simulink model "Pay_load"  (R2025a)
settings: Solver=ode4  StartTime=0.0  StopTime=1  FixedStep=0.001  RelTol=1e-3
values from neighbouring files (symbols this model uses):
  angle1_init = [0;0;0.3]    [param.m]
  angle2_init = [0;0;0.3]    [param.m]
  angle3_init = [0;0;0.3]    [param.m]
  angle4_init = [0;0;0.3]    [param.m]
  joint_matrix = [r1; r2; r3; r4]    [param.m]
  m1 = 1    [param.m]
  m2 = 1    [param.m]
  m3 = 1    [param.m]
  m4 = 1    [param.m]
  mL = 2    [param.m]
  P = block.DialogPrm(1).Data    [Load_dynamic.m]    (also in param.m = struct())
  p1_init = pL_init + RL_init*r1 - l1*e1    [param.m]
  p2_init = pL_init + RL_init*r2 - l2*e2    [param.m]
  p3_init = pL_init + RL_init*r3 - l3*e3    [param.m]
  p4_init = pL_init + RL_init*r4 - l4*e4    [param.m]
  r1 = [ 0.25; -0.20; -0.45]    [param.m]
  r2 = [-0.50; -0.40; -0.15]    [param.m]
  r3 = [-0.50;  0.40;  0.15]    [param.m]
  r4 = [ 0.50;  0.40;  0.00]    [param.m]
  xL_init = [pL_init; vL_init; angle_L_init; omega_L_init]    [param.m]
(part 2 of 3)

== matlab function Pay_load/PayLoad Controller/Subsystem/Adaptive Law (eq. 31) ==
  data: z4L input; delta_2L_dot output; delta_2L input
function delta_2L_dot = fcn(z4L, delta_2L)

    n_delta2L = 0.25; sigma_delta2L = 0.1; epsilon_L = 0.1;

    delta_2L_dot = n_delta2L*norm(z4L)^2/sqrt(norm(z4L)^2 + epsilon_L^2) - sigma_delta2L*delta_2L;

end

== matlab function Pay_load/PayLoad Controller/MATLAB Function3 ==
  data: angle_dL input; R_dL output
function R_dL = fcn(angle_dL)

    phi_dL = angle_dL(1); theta_dL = angle_dL(2); psi_dL = angle_dL(3);

    R_dL = [cos(theta_dL)*cos(psi_dL), sin(phi_dL)*sin(theta_dL)*cos(psi_dL) - cos(phi_dL)*sin(psi_dL), cos(phi_dL)*sin(theta_dL)*cos(psi_dL) + sin(phi_dL)*sin(psi_dL);
            cos(theta_dL)*sin(psi_dL), sin(phi_dL)*sin(theta_dL)*sin(psi_dL) + cos(phi_dL)*cos(psi_dL), cos(phi_dL)*sin(theta_dL)*sin(psi_dL) - sin(phi_dL)*cos(psi_dL);
            -sin(theta_dL)           , sin(phi_dL)*cos(theta_dL)                                      , cos(phi_dL)*cos(theta_dL)];

    
end

== matlab function Pay_load/PayLoad Controller/Equation (35) ==
  data: u input; cable_tension output; joint_matrix parameter
function cable_tension = fcn(u, joint_matrix)

    r1 = joint_matrix(1:3, 1);
    r2 = joint_matrix(4:6, 1);
    r3 = joint_matrix(7:9, 1);
    r4 = joint_matrix(10:12, 1);


    S = @(r) [0, -r(3), r(2);
              r(3), 0, -r(1);
              -r(2), r(1), 0];

    P = [eye(3), eye(3), eye(3), eye(3);
         S(r1) , S(r2) , S(r3) , S(r4)];

    P_inv = P' / (P * P');

    cable_tension = P_inv * u;

end

== matlab function Pay_load/PayLoad Controller/Equation (77) ==
  data: angle_L_dot input; Psi_L input; Psi_L_dot input; alpha_angle_L_dot input; alpha_angle_L input; sq_L output
function sq_L = fcn(angle_L_dot, Psi_L, Psi_L_dot, alpha_angle_L_dot, alpha_angle_L)

    S = @(r) [0, -r(3), r(2);
              r(3), 0, -r(1);
              -r(2), r(1), 0];
    
    sq_L = norm(Psi_L)*(norm(Psi_L*alpha_angle_L_dot + Psi_L_dot*alpha_angle_L) + norm(S(Psi_L*angle_L_dot))*norm(Psi_L*alpha_angle_L));

end

== matlab function Pay_load/UAV1 Controller/Subsystem1/Position Controller/Equation (8) ==
  data: ei input; dei output
function dei = fcn(ei)

    dei = norm(ei);

end

== matlab function Pay_load/Subsystem/UAV1/MATLAB Function ==
  data: a_free input; p_ddot output; fCableWorld input; m parameter
function p_ddot = UAV_Acceleration(a_free, fCableWorld, m)
%#codegen
% fCableWorld: luc day THUC tac dung len UAV, he the gioi.

assert(m > 0);

p_ddot = a_free + fCableWorld/m;
end

== matlab function Pay_load/UAV1 Controller/Subsystem1/Position Controller/Equation (15) ==
  data: dei input; eta_e1 output; t input; d_eta_d_dei output
function [eta_e1, d_eta_d_dei]= fcn(dei, t)
    
    eta_e1 = 0;

    Omega_dHi = (7.8 - 0.2)*exp(-0.4*t) + 0.2;

    eta_e1 = (Omega_dHi*dei)/(Omega_dHi - dei);

    d_eta_d_dei = Omega_dHi^2/(Omega_dHi - dei)^2;

end

== matlab function Pay_load/UAV1 Controller/Subsystem1/Position Controller/MATLAB Function ==
  data: dij input; t input; d_eij output; vij input; eta_eij output; d_eta_d_deij output
function [d_eij, eta_eij, d_eta_d_deij]   = fcn(dij, t, vij)

    d_eij = zeros(3,1);
    eta_eij = zeros(3,1);
    d_eta_d_deij = zeros(3,1);

    d12 = dij(1); d13 = dij(2); d14 = dij(3);
    v12 = vij(1); v13 = vij(2); v14 = vij(3);


    Omega_Hij = (2 - 0.1)*exp(-0.1*t) + 0.1;
    Omega_Wij = (1.8 - 0.1)*exp(-0.15*t) + 0.1;

    A = @(d_eij) (Omega_Hij*Omega_Wij*(Omega_Hij*Omega_Wij + d_eij^2))/((Omega_Hij - d_eij)^2*(Omega_Wij + d_eij)^2);

    d_e12 = d12 - v12; d_e13 = d13 - v13; d_e14 = d14 - v14;

    eta_e12 = (Omega_Hij*Omega_Wij*d_e12)/((Omega_Hij - d_e12) * (Omega_Wij + d_e12));
    eta_e13 = (Omega_Hij*Omega_Wij*d_e13)/((Omega_Hij - d_e13) * (Omega_Wij + d_e13));
    eta_e14 = (Omega_Hij*Omega_Wij*d_e14)/((Omega_Hij - d_e14) * (Omega_Wij + d_e14));

    d_eij = [d_e12; d_e13; d_e14];
    eta_eij = [eta_e12; eta_e13; eta_e14];

    d_eta_d_de12 = A(d_e12); d_eta_d_de13 = A(d_e13); d_eta_d_de14 = A(d_e14);

    d_eta_d_deij = [d_eta_d_de12; d_eta_d_de13; d_eta_d_de14];
    
end

== matlab function Pay_load/UAV1 Controller/Subsystem1/Position Controller/Equation (10) ==
  data: e12 input; dij output; e13 input; e14 input
function dij = fcn(e12, e13, e14)

    dij = zeros(3,1);

    d12 = norm(e12);
    d13 = norm(e13);
    d14 = norm(e14);


    dij = [d12; d13; d14];
end

== matlab function Pay_load/UAV1 Controller/Subsystem1/Position Controller/Equation (9) ==
  data: e_d12 input; vij output; e_d13 input; e_d14 input
function vij = fcn(e_d12, e_d13, e_d14)

    vij = zeros(3,1);

    v12 = norm(e_d12);
    v13 = norm(e_d13);
    v14 = norm(e_d14);

    vij = [v12; v13; v14];

end

== matlab function Pay_load/Subsystem/UAV1/MATLAB Function2 ==
  data: angle input; angle_dot output; omega input
function angle_dot = fcn(angle, omega)

    angle_dot = zeros(3,1);

    phi = angle(1); theta = angle(2);

    Gamma = [1, sin(phi)*tan(theta), cos(phi)*tan(theta);
            0, cos(phi), -sin(phi);
            0, sin(phi)/cos(theta), cos(phi)/cos(theta)];

    angle_dot = Gamma * omega;

end

== matlab function Pay_load/Subsystem1/UAV2/MATLAB Function2 ==
  data: angle input; angle_dot output; omega input
function angle_dot = fcn(angle, omega)

    angle_dot = zeros(3,1);

    phi = angle(1); theta = angle(2);

    Gamma = [1, sin(phi)*tan(theta), cos(phi)*tan(theta);
            0, cos(phi), -sin(phi);
            0, sin(phi)/cos(theta), cos(phi)/cos(theta)];

    angle_dot = Gamma * omega;

end

== matlab function Pay_load/Subsystem2/UAV3/MATLAB Function2 ==
  data: angle input; angle_dot output; omega input
function angle_dot = fcn(angle, omega)

    angle_dot = zeros(3,1);

    phi = angle(1); theta = angle(2);

    Gamma = [1, sin(phi)*tan(theta), cos(phi)*tan(theta);
            0, cos(phi), -sin(phi);
            0, sin(phi)/cos(theta), cos(phi)/cos(theta)];

    angle_dot = Gamma * omega;

end

== matlab function Pay_load/Subsystem3/UAV4/MATLAB Function2 ==
  data: angle input; angle_dot output; omega input
function angle_dot = fcn(angle, omega)

    angle_dot = zeros(3,1);

    phi = angle(1); theta = angle(2);

    Gamma = [1, sin(phi)*tan(theta), cos(phi)*tan(theta);
            0, cos(phi), -sin(phi);
            0, sin(phi)/cos(theta), cos(phi)/cos(theta)];

    angle_dot = Gamma * omega;

end

== matlab function Pay_load/UAV1 Controller/Subsystem1/Position Controller/MATLAB Function1 ==
  data: dei input; eta_ei input; d_eta_d_dei input; ei input; eij input; d_ij input; Ei output; eta_eij input; d_eta_d_eij input
function Ei = fcn(dei, eta_ei, d_eta_d_dei, ei, eij, d_ij, eta_eij, d_eta_d_eij)

    Ei = zeros(3,1);

    A = d_eta_d_dei * sqrt(d_eta_d_dei) * ei;
    
    B = zeros(3,1);
    for i = 1:3
        B = B + 2*eta_eij(i)*d_eta_d_eij(i)*eij(((i-1)*3+1):(i*3),1)/d_ij(i);
    end

    Ei = A + B;

end

== matlab function Pay_load/UAV1 Controller/Subsystem1/Position Controller/Equation (38) ==
  data: ei input; dei input; eta_ei input; d_eta_d_dei input; alpha_pi output; Ei input; eta_eij input; pd_dot input; t input; e_dij input; e_dij_dot input; vij input; d_eij input; d_eta_d_deij input
function alpha_pi = fcn(ei, dei, eta_ei, d_eta_d_dei, Ei, eta_eij, pd_dot, t, e_dij, e_dij_dot, vij, d_eij, d_eta_d_deij)

    alpha_pi = zeros(3,1);

    Kei = 3.15; Keij = 0.45;
    
    %% Eta_i
    Omega_dHi = (7.8 - 0.2)*exp(-0.4*t) + 0.2;
    Omega_dHi_dot = -0.4*7.6*exp(-0.4*t);
    d_eta_d_Omega_dHi = -dei^2/(Omega_dHi - dei)^2;

    h = Omega_dHi;
    hdot = Omega_dHi_dot;
    gap = h - dei;

    assert(gap > 1e-9, ...
        'Sai so vi tri da cham hoac vuot bien.');

    Gi = (h/gap)^3 * ei;

    eta_Eta_i = Gi.'*pd_dot ...
                + eta_ei*(dei^2/gap^2)*hdot;
    
    
    %% Eta_eij
    Omega_Hij = (2 - 0.1)*exp(-0.1*t) + 0.1;
    Omega_Wij = (1.8 - 0.1)*exp(-0.15*t) + 0.1;

    Omega_Hij_dot = -0.1*1.9*exp(-0.1*t);
    Omega_Wij_dot = -0.15*1.7*exp(-0.15*t);

    C_Hij = @(d_eij) -Omega_Wij*d_eij^2/((Omega_Hij - d_eij)^2 * (Omega_Wij + d_eij));
    D_Wij = @(d_eij) Omega_Hij*d_eij^2/((Omega_Hij - d_eij)*(Omega_Wij + d_eij)^2);

    d_eta_d_Omega_Hij = [C_Hij(d_eij(1)); C_Hij(d_eij(2)); C_Hij(d_eij(3))];
    d_eta_d_Omega_Wij = [D_Wij(d_eij(1)); D_Wij(d_eij(2)); D_Wij(d_eij(3))];


    e_d12 = e_dij(1:3,1); e_d13 = e_dij(4:6,1); e_d14 = e_dij(7:9,1);
    e_d12_dot = e_dij_dot(1:3,1); e_d13_dot = e_dij_dot(4:6,1); e_d14_dot = e_dij_dot(7:9,1);
    
    Eta_e12 = d_eta_d_deij(1)/vij(1)*(e_d12(1)*e_d12_dot(1) + e_d12(2)*e_d12_dot(2) + e_d12(3)*e_d12_dot(3)) - (d_eta_d_Omega_Hij(1)*Omega_Hij_dot + d_eta_d_Omega_Wij(1)*Omega_Wij_dot);
    Eta_e13 = d_eta_d_deij(2)/vij(2)*(e_d13(1)*e_d13_dot(1) + e_d13(2)*e_d13_dot(2) + e_d13(3)*e_d13_dot(3)) - (d_eta_d_Omega_Hij(2)*Omega_Hij_dot + d_eta_d_Omega_Wij(2)*Omega_Wij_dot);
    Eta_e14 = d_eta_d_deij(3)/vij(3)*(e_d14(1)*e_d14_dot(1) + e_d14(2)*e_d14_dot(2) + e_d14(3)*e_d14_dot(3)) - (d_eta_d_Omega_Hij(3)*Omega_Hij_dot + d_eta_d_Omega_Wij(3)*Omega_Wij_dot);

    Eta_eij = [Eta_e12; Eta_e13; Eta_e14];

    B = 0;
    for i = 1:3
        B = B - Keij*eta_eij(i)^2 + eta_eij(i)*Eta_eij(i);
    end

    den = Ei.'*Ei;

    assert(den > 1e-12, ...
        'Phuong trinh 38 gan ky di: Ei gan bang 0.');

    alpha_pi = Ei/den * ...
            (-Kei*eta_ei^2 + eta_Eta_i + B);

end

== matlab function Pay_load/Subsystem1/UAV2/MATLAB Function ==
  data: a_free input; p_ddot output; fCableWorld input; m parameter
function p_ddot = UAV_Acceleration(a_free, fCableWorld, m)
%#codegen
% fCableWorld: luc day THUC tac dung len UAV, he the gioi.

assert(m > 0);

p_ddot = a_free + fCableWorld/m;
end

== matlab function Pay_load/UAV1 Controller/Subsystem1/Subsystem/MATLAB Function ==
  data: pi input; vi input; ui output; alpha_pi input; alpha_pi_dot input; Ei input; cable_tension input; delta_i input; rho_mi input; xL input; z2i output; ubar_i output; delta_i_dot output; rho_mi_dot output; m parameter; ri parameter
function [ui, z2i, ubar_i, delta_i_dot, rho_mi_dot] = ...
    Velocity_Control_41_44(pi, vi, alpha_pi, alpha_pi_dot, Ei, ...
                          cable_tension, delta_i, rho_mi, xL, m, ri)
    %#codegen
    % Vector inputs: 3x1
    % mi, delta_i, rho_mi: scalar
    
    K2i       = 3.15;
    epsilon_i = 0.1;
    
    n_delta     = 0.15;
    sigma_delta = 0.05;
    
    n_rho_m     = 0.1;
    sigma_rho_m = 0.01;
    
    assert(m > 0);
    
    ez = [0; 0; 1];
    
    z2i = vi - alpha_pi;
    z2_sq = z2i.' * z2i;
    
    %% Equation (42)
    pL = xL(1:3,1); phi_L = xL(7,1); theta_L = xL(8,1); psi_L = xL(9,1);

    RL = [cos(theta_L)*cos(psi_L), sin(phi_L)*sin(theta_L)*cos(psi_L) - cos(phi_L)*sin(psi_L), cos(phi_L)*sin(theta_L)*cos(psi_L) + sin(phi_L)*sin(psi_L);
          cos(theta_L)*sin(psi_L), sin(phi_L)*sin(theta_L)*sin(psi_L) + cos(phi_L)*cos(psi_L), cos(phi_L)*sin(theta_L)*sin(psi_L) - sin(phi_L)*cos(psi_L);
          -sin(theta_L), sin(phi_L)*cos(theta_L), cos(phi_L)*cos(theta_L)];

    qi = RL.'*(pL + RL*ri - pi)/norm(pL + RL*ri - pi);

    fCablePred_i = RL*qi*(cable_tension.'*qi);

    ubar_i = Ei - alpha_pi_dot ...
             + 9.81 * ez ...
             + K2i * z2i ...
             + delta_i * z2i / sqrt(z2_sq + epsilon_i^2) ...
             + fCablePred_i / m;
    
    %% Equation (41)
    ubar_sq = ubar_i.' * ubar_i;
    A = ubar_sq * rho_mi^2;
    
    ui = z2i * A / sqrt(z2_sq * A + epsilon_i^2);
    
    %% Equation (43)
    delta_i_dot = n_delta * z2_sq ...
                  / sqrt(z2_sq + epsilon_i^2) ...
                  - sigma_delta * delta_i;
    
    %% Equation (44)
    rho_mi_dot = n_rho_m * (z2i.' * ubar_i) ...
                - sigma_rho_m * rho_mi;

end

== matlab function Pay_load/UAV1 Controller/Subsystem1/Subsystem/MATLAB Function1 ==
  data: ui input; Fi output; psi_di input; angle_di_prev input; angle_di output; valid output
function [Fi, angle_di, valid] = ...
    Desired_Attitude_85_87(ui, psi_di, angle_di_prev)
%#codegen
% ui, angle_di_prev: 3x1
% psi_di, Fi: scalar
% valid: boolean

Fmin = 1e-8;

Fi = norm(ui);
angle_di = angle_di_prev;
valid = false;

% Khi ui gan 0, huong luc khong xac dinh.
% Giu goc dat truoc do, khong chia cho Fi.
if Fi <= Fmin
    return;
end

% Mien Euler bay thang dang su dung:
% |phi_di| < pi/2, |theta_di| < pi/2.
% assert(ui(3) > 0);

sphi = (ui(1)*sin(psi_di) ...
        - ui(2)*cos(psi_di)) / Fi;

% Chi chan sai so lam tron cua asin.
sphi = min(1.0, max(-1.0, sphi));

phi_di = asin(sphi);

theta_di = atan2( ...
    ui(1)*cos(psi_di) + ui(2)*sin(psi_di), ui(3));

angle_di = [phi_di; theta_di; psi_di];
valid = true;

end

== matlab function Pay_load/UAV1 Controller/Subsystem/MATLAB Function ==
  data: angle_i input; z3i output size=[3,1]; omega_i input; angle_di input; z4i output size=[3,1]; Gamma_i output size=[3,3]; alpha_angle_i output size=[3,1]; angle_i_dot output size=[3,1]; Psi_i output size=[3,3]; Psi_i_dot output size=[3,3]
function [z3i, z4i, Gamma_i, alpha_angle_i, angle_i_dot, Psi_i, Psi_i_dot] = ...
    Attitude_Error_56(angle_i, omega_i, angle_di)


    z3i = zeros(3,1);
    z4i = zeros(3,1);

    Gamma_i = zeros(3,3);

    alpha_angle_i = zeros(3,1);

    K3i = 0.75;
    nu_i = 0.5;
    
    phi   = angle_i(1);
    theta = angle_i(2);
    
    sp = sin(phi);
    cp = cos(phi);
    st = sin(theta);
    ct = cos(theta);
    
    assert(K3i > 0 && nu_i > 0);
    assert(abs(ct) > 1e-6);
    
    Gamma_i = [1, sp*st/ct, cp*st/ct;
               0, cp,       -sp;
               0, sp/ct,    cp/ct];
    
    Psi_i = [1, 0,   -st;
             0, cp,  sp*ct;
             0, -sp, cp*ct];
    
    angle_i_dot = Gamma_i * omega_i;
    
    z3i = angle_i - angle_di;
    
    k = K3i + 0.5*nu_i;
    alpha_angle_i = -k * z3i;
    
    z4i = angle_i_dot - alpha_angle_i;
    
    % Dao ham giai tich cua Psi_i
    phi_dot   = angle_i_dot(1);
    theta_dot = angle_i_dot(2);
    
    Psi_i_dot = ...
        [0, 0, -ct*theta_dot;
         0, -sp*phi_dot, ...
            cp*ct*phi_dot - sp*st*theta_dot;
         0, -cp*phi_dot, ...
            -sp*ct*phi_dot - cp*st*theta_dot];

end

== matlab function Pay_load/UAV1 Controller/Subsystem/MATLAB Function1 ==
  data: alpha_angle_i input; angle_i_dot input; Psi_i input; Xi_i output; Psi_i_dot input
function Xi_i = Xi_89(alpha_angle_i, angle_i_dot, Psi_i, Psi_i_dot)

    Xi_i = 0;

    K3i = 0.75; nu_i = 0.5;
    
    k = K3i + 0.5*nu_i;
    
    w = Psi_i * angle_i_dot;
    
    S_w = [0,    -w(3),  w(2);
           w(3),  0,    -w(1);
          -w(2),  w(1),  0];
    
    term1 = norm(Psi_i_dot * alpha_angle_i);
    term2 = norm(k * Psi_i * angle_i_dot);
    term3 = norm(S_w, 2) * norm(Psi_i * alpha_angle_i);
    term4 = norm(k * Psi_i, 2);
    
    Xi_i = norm(Psi_i, 2) * (term1 + term2 + term3 + term4);

end

== matlab function Pay_load/UAV1 Controller/Subsystem/MATLAB Function2 ==
  data: z3i input; tau_i output; z4i input; Gamma_i input; Psi_i input; Xi_i input; rho_Ji input; zeta_i input; tau_bar_i output; rho_Ji_dot output; zeta_i_dot output
function [tau_i, tau_bar_i, rho_Ji_dot, zeta_i_dot] = ...
    Torque_Control_58_61(z3i, z4i, Gamma_i, Psi_i, ...
                         Xi_i, rho_Ji, zeta_i)
%#codegen
% z3i, z4i, tau_i, tau_bar_i: 3x1
% Gamma_i, Psi_i: 3x3
% Other inputs and adaptive derivatives: scalar

epsilon_i = 0.1;

n_rho_J     = 0.15;
sigma_rho_J = 0.05;

n_zeta     = 0.15;
sigma_zeta = 0.05;

K4i = 0.75;

assert(K4i > 0);

z4_sq = z4i.' * z4i;
Xi_sq = Xi_i^2;

den_zeta = sqrt(z4_sq * Xi_sq + epsilon_i^2);

% Equation (59)
GammaT_z4 = Gamma_i.' * z4i;

tau_bar_i = K4i * GammaT_z4 ...
            + Gamma_i.' * z3i ...
            + zeta_i * GammaT_z4 * Xi_sq / den_zeta;

% Equation (58)
q = Psi_i * z4i;

tau_bar_sq = tau_bar_i.' * tau_bar_i;
A = tau_bar_sq * rho_Ji^2;

tau_i = -q * A / sqrt((q.' * q) * A + epsilon_i^2);

% Equation (60)
rho_Ji_dot = n_rho_J * (q.' * tau_bar_i) ...
            - sigma_rho_J * rho_Ji;

% Equation (61)
zeta_i_dot = n_zeta * z4_sq * Xi_sq / den_zeta ...
            - sigma_zeta * zeta_i;

end

== matlab function Pay_load/UAV2 Controller/Subsystem/MATLAB Function ==
  data: angle_i input; z3i output size=[3,1]; omega_i input; angle_di input; z4i output size=[3,1]; Gamma_i output size=[3,3]; alpha_angle_i output size=[3,1]; angle_i_dot output size=[3,1]; Psi_i output size=[3,3]; Psi_i_dot output size=[3,3]
function [z3i, z4i, Gamma_i, alpha_angle_i, angle_i_dot, Psi_i, Psi_i_dot] = ...
    Attitude_Error_56(angle_i, omega_i, angle_di)


    K3i = 0.75;
    nu_i = 0.5;
    
    phi   = angle_i(1);
    theta = angle_i(2);
    
    sp = sin(phi);
    cp = cos(phi);
    st = sin(theta);
    ct = cos(theta);
    
    assert(K3i > 0 && nu_i > 0);
    assert(abs(ct) > 1e-6);
    
    Gamma_i = [1, sp*st/ct, cp*st/ct;
               0, cp,       -sp;
               0, sp/ct,    cp/ct];
    
    Psi_i = [1, 0,   -st;
             0, cp,  sp*ct;
             0, -sp, cp*ct];
    
    angle_i_dot = Gamma_i * omega_i;
    
    z3i = angle_i - angle_di;
    
    k = K3i + 0.5*nu_i;
    alpha_angle_i = -k * z3i;
    
    z4i = angle_i_dot - alpha_angle_i;
    
    % Dao ham giai tich cua Psi_i
    phi_dot   = angle_i_dot(1);
    theta_dot = angle_i_dot(2);
    
    Psi_i_dot = ...
        [0, 0, -ct*theta_dot;
         0, -sp*phi_dot, ...
            cp*ct*phi_dot - sp*st*theta_dot;
         0, -cp*phi_dot, ...
            -sp*ct*phi_dot - cp*st*theta_dot];

end

== matlab function Pay_load/Subsystem/UAV1/MATLAB Function1 ==
  data: tau input; omega_dot output; omega input; Iv parameter
function omega_dot = fcn(tau, omega, Iv)

    omega_dot = zeros(3,1);

    omega_dot = Iv \ (tau - cross(omega, Iv*omega));

end

== matlab function Pay_load/UAV2 Controller/Subsystem/MATLAB Function1 ==
  data: alpha_angle_i input; angle_i_dot input; Psi_i input; Xi_i output size=1; Psi_i_dot input
function Xi_i = Xi_89(alpha_angle_i, angle_i_dot, Psi_i, Psi_i_dot)

K3i = 0.75; nu_i = 0.5;

k = K3i + 0.5*nu_i;

w = Psi_i * angle_i_dot;

S_w = [0,    -w(3),  w(2);
       w(3),  0,    -w(1);
      -w(2),  w(1),  0];

term1 = norm(Psi_i_dot * alpha_angle_i);
term2 = norm(k * Psi_i * angle_i_dot);
term3 = norm(S_w, 2) * norm(Psi_i * alpha_angle_i);
term4 = norm(k * Psi_i, 2);

Xi_i = norm(Psi_i, 2) * (term1 + term2 + term3 + term4);

end

== matlab function Pay_load/UAV2 Controller/Subsystem/MATLAB Function2 ==
  data: z3i input; tau_i output; z4i input; Gamma_i input; Psi_i input; Xi_i input; rho_Ji input; zeta_i input; tau_bar_i output; rho_Ji_dot output; zeta_i_dot output
function [tau_i, tau_bar_i, rho_Ji_dot, zeta_i_dot] = ...
    Torque_Control_58_61(z3i, z4i, Gamma_i, Psi_i, ...
                         Xi_i, rho_Ji, zeta_i)
%#codegen
% z3i, z4i, tau_i, tau_bar_i: 3x1
% Gamma_i, Psi_i: 3x3
% Other inputs and adaptive derivatives: scalar

epsilon_i = 0.1;

n_rho_J     = 0.15;
sigma_rho_J = 0.05;

n_zeta     = 0.15;
sigma_zeta = 0.05;

K4i = 0.75;

assert(K4i > 0);

z4_sq = z4i.' * z4i;
Xi_sq = Xi_i^2;

den_zeta = sqrt(z4_sq * Xi_sq + epsilon_i^2);

% Equation (59)
GammaT_z4 = Gamma_i.' * z4i;

tau_bar_i = K4i * GammaT_z4 ...
            + Gamma_i.' * z3i ...
            + zeta_i * GammaT_z4 * Xi_sq / den_zeta;

% Equation (58)
q = Psi_i * z4i;

tau_bar_sq = tau_bar_i.' * tau_bar_i;
A = tau_bar_sq * rho_Ji^2;

tau_i = -q * A / sqrt((q.' * q) * A + epsilon_i^2);

% Equation (60)
rho_Ji_dot = n_rho_J * (q.' * tau_bar_i) ...
            - sigma_rho_J * rho_Ji;

% Equation (61)
zeta_i_dot = n_zeta * z4_sq * Xi_sq / den_zeta ...
            - sigma_zeta * zeta_i;

end

== matlab function Pay_load/UAV2 Controller/Subsystem1/Position Controller/Equation (10) ==
  data: e21 input; dij output; e23 input; e24 input
function dij = fcn(e21, e23, e24)

    dij = zeros(3,1);

    d21 = norm(e21);
    d23 = norm(e23);
    d24 = norm(e24);


    dij = [d21; d23; d24];
end

== matlab function Pay_load/UAV2 Controller/Subsystem1/Position Controller/Equation (15) ==
  data: dei input; eta_e2 output; t input; d_eta_d_dei output
function [eta_e2, d_eta_d_dei]= fcn(dei, t)
    
    eta_e1 = 0;

    Omega_dHi = (7.8 - 0.2)*exp(-0.4*t) + 0.2;

    eta_e2 = (Omega_dHi*dei)/(Omega_dHi - dei);

    d_eta_d_dei = Omega_dHi^2/(Omega_dHi - dei)^2;

end

== matlab function Pay_load/UAV2 Controller/Subsystem1/Position Controller/Equation (38) ==
  data: ei input; dei input; eta_ei input; d_eta_d_dei input; alpha_pi output; Ei input; eta_eij input; pd_dot input; t input; e_dij input; e_dij_dot input; vij input; d_eij input; d_eta_d_deij input
function alpha_pi = fcn(ei, dei, eta_ei, d_eta_d_dei, Ei, eta_eij, pd_dot, t, e_dij, e_dij_dot, vij, d_eij, d_eta_d_deij)

    alpha_pi = zeros(3,1);

    Kei = 3.15; Keij = 0.45;
    
    %% Eta_i
    Omega_dHi = (7.8 - 0.2)*exp(-0.4*t) + 0.2;
    Omega_dHi_dot = -0.4*7.6*exp(-0.4*t);
    d_eta_d_Omega_dHi = -dei^2/(Omega_dHi - dei)^2;

    h = Omega_dHi;
    hdot = Omega_dHi_dot;
    gap = h - dei;

    assert(gap > 1e-9, ...
        'Sai so vi tri da cham hoac vuot bien.');

    Gi = (h/gap)^3 * ei;

    eta_Eta_i = Gi.'*pd_dot ...
                + eta_ei*(dei^2/gap^2)*hdot;
    
    
    %% Eta_eij
    Omega_Hij = (2 - 0.1)*exp(-0.1*t) + 0.1;
    Omega_Wij = (1.8 - 0.1)*exp(-0.15*t) + 0.1;

    Omega_Hij_dot = -0.1*1.9*exp(-0.1*t);
    Omega_Wij_dot = -0.15*1.7*exp(-0.15*t);

    C_Hij = @(d_eij) -Omega_Wij*d_eij^2/((Omega_Hij - d_eij)^2 * (Omega_Wij + d_eij));
    D_Wij = @(d_eij) Omega_Hij*d_eij^2/((Omega_Hij - d_eij)*(Omega_Wij + d_eij)^2);

    d_eta_d_Omega_Hij = [C_Hij(d_eij(1)); C_Hij(d_eij(2)); C_Hij(d_eij(3))];
    d_eta_d_Omega_Wij = [D_Wij(d_eij(1)); D_Wij(d_eij(2)); D_Wij(d_eij(3))];


    e_d12 = e_dij(1:3,1); e_d13 = e_dij(4:6,1); e_d14 = e_dij(7:9,1);
    e_d12_dot = e_dij_dot(1:3,1); e_d13_dot = e_dij_dot(4:6,1); e_d14_dot = e_dij_dot(7:9,1);
    
    Eta_e12 = d_eta_d_deij(1)/vij(1)*(e_d12(1)*e_d12_dot(1) + e_d12(2)*e_d12_dot(2) + e_d12(3)*e_d12_dot(3)) - (d_eta_d_Omega_Hij(1)*Omega_Hij_dot + d_eta_d_Omega_Wij(1)*Omega_Wij_dot);
    Eta_e13 = d_eta_d_deij(2)/vij(2)*(e_d13(1)*e_d13_dot(1) + e_d13(2)*e_d13_dot(2) + e_d13(3)*e_d13_dot(3)) - (d_eta_d_Omega_Hij(2)*Omega_Hij_dot + d_eta_d_Omega_Wij(2)*Omega_Wij_dot);
    Eta_e14 = d_eta_d_deij(3)/vij(3)*(e_d14(1)*e_d14_dot(1) + e_d14(2)*e_d14_dot(2) + e_d14(3)*e_d14_dot(3)) - (d_eta_d_Omega_Hij(3)*Omega_Hij_dot + d_eta_d_Omega_Wij(3)*Omega_Wij_dot);

    Eta_eij = [Eta_e12; Eta_e13; Eta_e14];

    B = 0;
    for i = 1:3
        B = B - Keij*eta_eij(i)^2 + eta_eij(i)*Eta_eij(i);
    end

    den = Ei.'*Ei;

    assert(den > 1e-12, ...
        'Phuong trinh 38 gan ky di: Ei gan bang 0.');

    alpha_pi = Ei/den * ...
            (-Kei*eta_ei^2 + eta_Eta_i + B);

end

== matlab function Pay_load/UAV2 Controller/Subsystem1/Position Controller/Equation (8) ==
  data: ei input; dei output
function dei = fcn(ei)

    dei = norm(ei);

end

== matlab function Pay_load/UAV2 Controller/Subsystem1/Position Controller/Equation (9) ==
  data: e_d21 input; vij output; e_d23 input; e_d24 input
function vij = fcn(e_d21, e_d23, e_d24)

    vij = zeros(3,1);

    v21 = norm(e_d21);
    v23 = norm(e_d23);
    v24 = norm(e_d24);

    vij = [v21; v23; v24];

end

== matlab function Pay_load/Subsystem1/UAV2/MATLAB Function1 ==
  data: tau input; omega_dot output; omega input; Iv parameter
function omega_dot = fcn(tau, omega, Iv)

    omega_dot = zeros(3,1);

    omega_dot = Iv \ (tau - cross(omega, Iv*omega));

end

== matlab function Pay_load/UAV2 Controller/Subsystem1/Position Controller/MATLAB Function ==
  data: dij input; t input; d_eij output; vij input; eta_eij output; d_eta_d_deij output
function [d_eij, eta_eij, d_eta_d_deij]   = fcn(dij, t, vij)

    d_eij = zeros(3,1);
    eta_eij = zeros(3,1);
    d_eta_d_deij = zeros(3,1);

    d12 = dij(1); d13 = dij(2); d14 = dij(3);
    v12 = vij(1); v13 = vij(2); v14 = vij(3);


    Omega_Hij = (2 - 0.1)*exp(-0.1*t) + 0.1;
    Omega_Wij = (1.8 - 0.1)*exp(-0.15*t) + 0.1;

    A = @(d_eij) (Omega_Hij*Omega_Wij*(Omega_Hij*Omega_Wij + d_eij^2))/((Omega_Hij - d_eij)^2*(Omega_Wij + d_eij)^2);

    d_e12 = d12 - v12; d_e13 = d13 - v13; d_e14 = d14 - v14;

    eta_e12 = (Omega_Hij*Omega_Wij*d_e12)/((Omega_Hij - d_e12) * (Omega_Wij + d_e12));
    eta_e13 = (Omega_Hij*Omega_Wij*d_e13)/((Omega_Hij - d_e13) * (Omega_Wij + d_e13));
    eta_e14 = (Omega_Hij*Omega_Wij*d_e14)/((Omega_Hij - d_e14) * (Omega_Wij + d_e14));

    d_eij = [d_e12; d_e13; d_e14];
    eta_eij = [eta_e12; eta_e13; eta_e14];

    d_eta_d_de12 = A(d_e12); d_eta_d_de13 = A(d_e13); d_eta_d_de14 = A(d_e14);

    d_eta_d_deij = [d_eta_d_de12; d_eta_d_de13; d_eta_d_de14];
    
end

== matlab function Pay_load/UAV2 Controller/Subsystem1/Position Controller/MATLAB Function1 ==
  data: dei input; eta_ei input; d_eta_d_dei input; ei input; eij input; d_ij input; Ei output; eta_eij input; d_eta_d_eij input
function Ei = fcn(dei, eta_ei, d_eta_d_dei, ei, eij, d_ij, eta_eij, d_eta_d_eij)

    Ei = zeros(3,1);

    A = d_eta_d_dei * sqrt(d_eta_d_dei) * ei;
    
    B = zeros(3,1);
    for i = 1:3
        B = B + 2*eta_eij(i)*d_eta_d_eij(i)*eij(((i-1)*3+1):(i*3),1)/d_ij(i);
    end

    Ei = A + B;

end

== matlab function Pay_load/UAV2 Controller/Subsystem1/Subsystem/MATLAB Function ==
  data: pi input; vi input; ui output; alpha_pi input; alpha_pi_dot input; Ei input; cable_tension input; delta_i input; rho_mi input; xL input; z2i output; ubar_i output; delta_i_dot output; rho_mi_dot output; m parameter; ri parameter
function [ui, z2i, ubar_i, delta_i_dot, rho_mi_dot] = ...
    Velocity_Control_41_44(pi, vi, alpha_pi, alpha_pi_dot, Ei, ...
                          cable_tension, delta_i, rho_mi, xL, m, ri)
    %#codegen
    % Vector inputs: 3x1
    % mi, delta_i, rho_mi: scalar
    
    K2i       = 3.15;
    epsilon_i = 0.1;
    
    n_delta     = 0.15;
    sigma_delta = 0.05;
    
    n_rho_m     = 0.1;
    sigma_rho_m = 0.01;
    
    assert(m > 0);
    
    ez = [0; 0; 1];
    
    z2i = vi - alpha_pi;
    z2_sq = z2i.' * z2i;
    
    %% Equation (42)
    pL = xL(1:3,1); phi_L = xL(7,1); theta_L = xL(8,1); psi_L = xL(9,1);

    RL = [cos(theta_L)*cos(psi_L), sin(phi_L)*sin(theta_L)*cos(psi_L) - cos(phi_L)*sin(psi_L), cos(phi_L)*sin(theta_L)*cos(psi_L) + sin(phi_L)*sin(psi_L);
          cos(theta_L)*sin(psi_L), sin(phi_L)*sin(theta_L)*sin(psi_L) + cos(phi_L)*cos(psi_L), cos(phi_L)*sin(theta_L)*sin(psi_L) - sin(phi_L)*cos(psi_L);
          -sin(theta_L), sin(phi_L)*cos(theta_L), cos(phi_L)*cos(theta_L)];

    qi = RL.'*(pL + RL*ri - pi)/norm(pL + RL*ri - pi);

    fCablePred_i = RL*qi*(cable_tension.'*qi);

    ubar_i = Ei - alpha_pi_dot ...
             + 9.81 * ez ...
             + K2i * z2i ...
             + delta_i * z2i / sqrt(z2_sq + epsilon_i^2) ...
             + fCablePred_i / m;
    
    %% Equation (41)
    ubar_sq = ubar_i.' * ubar_i;
    A = ubar_sq * rho_mi^2;
    
    ui = z2i * A / sqrt(z2_sq * A + epsilon_i^2);
    
    %% Equation (43)
    delta_i_dot = n_delta * z2_sq ...
                  / sqrt(z2_sq + epsilon_i^2) ...
                  - sigma_delta * delta_i;
    
    %% Equation (44)
    rho_mi_dot = n_rho_m * (z2i.' * ubar_i) ...
                - sigma_rho_m * rho_mi;

end

== matlab function Pay_load/UAV2 Controller/Subsystem1/Subsystem/MATLAB Function1 ==
  data: ui input; Fi output; psi_di input; angle_di_prev input; angle_di output size=[3,1]; valid output
function [Fi, angle_di, valid] = ...
    Desired_Attitude_85_87(ui, psi_di, angle_di_prev)
%#codegen
% ui, angle_di_prev: 3x1
% psi_di, Fi: scalar
% valid: boolean

Fmin = 1e-8;

Fi = norm(ui);
angle_di = angle_di_prev;
valid = false;

% Khi ui gan 0, huong luc khong xac dinh.
% Giu goc dat truoc do, khong chia cho Fi.
if Fi <= Fmin
    return;
end

% Mien Euler bay thang dang su dung:
% |phi_di| < pi/2, |theta_di| < pi/2.
% assert(ui(3) > 0);

sphi = (ui(1)*sin(psi_di) ...
        - ui(2)*cos(psi_di)) / Fi;

% Chi chan sai so lam tron cua asin.
sphi = min(1.0, max(-1.0, sphi));

phi_di = asin(sphi);

theta_di = atan2( ...
    ui(1)*cos(psi_di) + ui(2)*sin(psi_di), ui(3));

angle_di = [phi_di; theta_di; psi_di];
valid = true;

end

== matlab function Pay_load/UAV3 Controller/Subsystem/MATLAB Function ==
  data: angle_i input size=[3,1]; z3i output size=[3,1]; omega_i input size=[3,1]; angle_di input size=[3,1]; z4i output size=[3,1]; Gamma_i output size=[3,3]; alpha_angle_i output size=[3,1]; angle_i_dot output size=[3,1]; Psi_i output size=[3,3]; Psi_i_dot output size=[3,3]
function [z3i, z4i, Gamma_i, alpha_angle_i, angle_i_dot, Psi_i, Psi_i_dot] = ...
    Attitude_Error_56(angle_i, omega_i, angle_di)


    K3i = 0.75;
    nu_i = 0.5;
    
    phi   = angle_i(1);
    theta = angle_i(2);
    
    sp = sin(phi);
    cp = cos(phi);
    st = sin(theta);
    ct = cos(theta);
    
    assert(K3i > 0 && nu_i > 0);
    assert(abs(ct) > 1e-6);
    
    Gamma_i = [1, sp*st/ct, cp*st/ct;
               0, cp,       -sp;
               0, sp/ct,    cp/ct];
    
    Psi_i = [1, 0,   -st;
             0, cp,  sp*ct;
             0, -sp, cp*ct];
    
    angle_i_dot = Gamma_i * omega_i;
    
    z3i = angle_i - angle_di;
    
    k = K3i + 0.5*nu_i;
    alpha_angle_i = -k * z3i;
    
    z4i = angle_i_dot - alpha_angle_i;
    
    % Dao ham giai tich cua Psi_i
    phi_dot   = angle_i_dot(1);
    theta_dot = angle_i_dot(2);
    
    Psi_i_dot = ...
        [0, 0, -ct*theta_dot;
         0, -sp*phi_dot, ...
            cp*ct*phi_dot - sp*st*theta_dot;
         0, -cp*phi_dot, ...
            -sp*ct*phi_dot - cp*st*theta_dot];

end

== matlab function Pay_load/UAV3 Controller/Subsystem/MATLAB Function1 ==
  data: alpha_angle_i input; angle_i_dot input; Psi_i input; Xi_i output size=1; Psi_i_dot input
function Xi_i = Xi_89(alpha_angle_i, angle_i_dot, Psi_i, Psi_i_dot)

K3i = 0.75; nu_i = 0.5;

k = K3i + 0.5*nu_i;

w = Psi_i * angle_i_dot;

S_w = [0,    -w(3),  w(2);
       w(3),  0,    -w(1);
      -w(2),  w(1),  0];

term1 = norm(Psi_i_dot * alpha_angle_i);
term2 = norm(k * Psi_i * angle_i_dot);
term3 = norm(S_w, 2) * norm(Psi_i * alpha_angle_i);
term4 = norm(k * Psi_i, 2);

Xi_i = norm(Psi_i, 2) * (term1 + term2 + term3 + term4);

end

== matlab function Pay_load/UAV3 Controller/Subsystem/MATLAB Function2 ==
  data: z3i input; tau_i output; z4i input; Gamma_i input; Psi_i input; Xi_i input; rho_Ji input; zeta_i input; tau_bar_i output; rho_Ji_dot output; zeta_i_dot output
function [tau_i, tau_bar_i, rho_Ji_dot, zeta_i_dot] = ...
    Torque_Control_58_61(z3i, z4i, Gamma_i, Psi_i, ...
                         Xi_i, rho_Ji, zeta_i)
%#codegen
% z3i, z4i, tau_i, tau_bar_i: 3x1
% Gamma_i, Psi_i: 3x3
% Other inputs and adaptive derivatives: scalar

epsilon_i = 0.1;

n_rho_J     = 0.15;
sigma_rho_J = 0.05;

n_zeta     = 0.15;
sigma_zeta = 0.05;

K4i = 0.75;

assert(K4i > 0);

z4_sq = z4i.' * z4i;
Xi_sq = Xi_i^2;

den_zeta = sqrt(z4_sq * Xi_sq + epsilon_i^2);

% Equation (59)
GammaT_z4 = Gamma_i.' * z4i;

tau_bar_i = K4i * GammaT_z4 ...
            + Gamma_i.' * z3i ...
            + zeta_i * GammaT_z4 * Xi_sq / den_zeta;

% Equation (58)
q = Psi_i * z4i;

tau_bar_sq = tau_bar_i.' * tau_bar_i;
A = tau_bar_sq * rho_Ji^2;

tau_i = -q * A / sqrt((q.' * q) * A + epsilon_i^2);

% Equation (60)
rho_Ji_dot = n_rho_J * (q.' * tau_bar_i) ...
            - sigma_rho_J * rho_Ji;

% Equation (61)
zeta_i_dot = n_zeta * z4_sq * Xi_sq / den_zeta ...
            - sigma_zeta * zeta_i;

end

== matlab function Pay_load/Subsystem2/UAV3/MATLAB Function ==
  data: a_free input; p_ddot output; fCableWorld input; m parameter
function p_ddot = UAV_Acceleration(a_free, fCableWorld, m)
%#codegen
% fCableWorld: luc day THUC tac dung len UAV, he the gioi.

assert(m > 0);

p_ddot = a_free + fCableWorld/m;
end

== matlab function Pay_load/UAV3 Controller/Subsystem1/Position Controller/Equation (10) ==
  data: e31 input; dij output; e32 input; e34 input
function dij = fcn(e31, e32, e34)

    dij = zeros(3,1);

    d31 = norm(e31);
    d32 = norm(e32);
    d34 = norm(e34);


    dij = [d31; d32; d34];
end

== matlab function Pay_load/UAV3 Controller/Subsystem1/Position Controller/Equation (15) ==
  data: dei input; eta_e3 output; t input; d_eta_d_dei output
function [eta_e3, d_eta_d_dei]= fcn(dei, t)
    
    eta_e3 = 0;

    Omega_dHi = (7.8 - 0.2)*exp(-0.4*t) + 0.2;

    eta_e3 = (Omega_dHi*dei)/(Omega_dHi - dei);

    d_eta_d_dei = Omega_dHi^2/(Omega_dHi - dei)^2;

end

== matlab function Pay_load/UAV3 Controller/Subsystem1/Position Controller/Equation (38) ==
  data: ei input; dei input; eta_ei input; d_eta_d_dei input; alpha_pi output; Ei input; eta_eij input; pd_dot input; t input; e_dij input; e_dij_dot input; vij input; d_eij input; d_eta_d_deij input; gap output
function [alpha_pi, gap]= fcn(ei, dei, eta_ei, d_eta_d_dei, Ei, eta_eij, pd_dot, t, e_dij, e_dij_dot, vij, d_eij, d_eta_d_deij)

    alpha_pi = zeros(3,1);

    Kei = 3.15; Keij = 0.45;
    
    %% Eta_i
    Omega_dHi = (7.8 - 0.2)*exp(-0.4*t) + 0.2;
    Omega_dHi_dot = -0.4*7.6*exp(-0.4*t);
    d_eta_d_Omega_dHi = -dei^2/(Omega_dHi - dei)^2;

    h = Omega_dHi;
    hdot = Omega_dHi_dot;
    gap = h - dei;

    assert(gap > 1e-9, ...
        'Sai so vi tri da cham hoac vuot bien.');

    Gi = (h/gap)^3 * ei;

    eta_Eta_i = Gi.'*pd_dot ...
                + eta_ei*(dei^2/gap^2)*hdot;
    
    
    %% Eta_eij
    Omega_Hij = (2 - 0.1)*exp(-0.1*t) + 0.1;
    Omega_Wij = (1.8 - 0.1)*exp(-0.15*t) + 0.1;

    Omega_Hij_dot = -0.1*1.9*exp(-0.1*t);
    Omega_Wij_dot = -0.15*1.7*exp(-0.15*t);

    C_Hij = @(d_eij) -Omega_Wij*d_eij^2/((Omega_Hij - d_eij)^2 * (Omega_Wij + d_eij));
    D_Wij = @(d_eij) Omega_Hij*d_eij^2/((Omega_Hij - d_eij)*(Omega_Wij + d_eij)^2);

    d_eta_d_Omega_Hij = [C_Hij(d_eij(1)); C_Hij(d_eij(2)); C_Hij(d_eij(3))];
    d_eta_d_Omega_Wij = [D_Wij(d_eij(1)); D_Wij(d_eij(2)); D_Wij(d_eij(3))];


    e_d12 = e_dij(1:3,1); e_d13 = e_dij(4:6,1); e_d14 = e_dij(7:9,1);
    e_d12_dot = e_dij_dot(1:3,1); e_d13_dot = e_dij_dot(4:6,1); e_d14_dot = e_dij_dot(7:9,1);
    
    Eta_e12 = d_eta_d_deij(1)/vij(1)*(e_d12(1)*e_d12_dot(1) + e_d12(2)*e_d12_dot(2) + e_d12(3)*e_d12_dot(3)) - (d_eta_d_Omega_Hij(1)*Omega_Hij_dot + d_eta_d_Omega_Wij(1)*Omega_Wij_dot);
    Eta_e13 = d_eta_d_deij(2)/vij(2)*(e_d13(1)*e_d13_dot(1) + e_d13(2)*e_d13_dot(2) + e_d13(3)*e_d13_dot(3)) - (d_eta_d_Omega_Hij(2)*Omega_Hij_dot + d_eta_d_Omega_Wij(2)*Omega_Wij_dot);
    Eta_e14 = d_eta_d_deij(3)/vij(3)*(e_d14(1)*e_d14_dot(1) + e_d14(2)*e_d14_dot(2) + e_d14(3)*e_d14_dot(3)) - (d_eta_d_Omega_Hij(3)*Omega_Hij_dot + d_eta_d_Omega_Wij(3)*Omega_Wij_dot);

    Eta_eij = [Eta_e12; Eta_e13; Eta_e14];

    B = 0;
    for i = 1:3
        B = B - Keij*eta_eij(i)^2 + eta_eij(i)*Eta_eij(i);
    end

    den = Ei.'*Ei;

    assert(den > 1e-12, ...
        'Phuong trinh 38 gan ky di: Ei gan bang 0.');

    alpha_pi = Ei/den * ...
            (-Kei*eta_ei^2 + eta_Eta_i + B);

end

== matlab function Pay_load/UAV3 Controller/Subsystem1/Position Controller/Equation (8) ==
  data: ei input; dei output
function dei = fcn(ei)

    dei = norm(ei);

end

== matlab function Pay_load/UAV3 Controller/Subsystem1/Position Controller/Equation (9) ==
  data: e_d31 input; vij output; e_d32 input; e_d34 input
function vij = fcn(e_d31, e_d32, e_d34)

    vij = zeros(3,1);

    v31 = norm(e_d31);
    v32 = norm(e_d32);
    v34 = norm(e_d34);

    vij = [v31; v32; v34];

end

== matlab function Pay_load/UAV3 Controller/Subsystem1/Position Controller/MATLAB Function ==
  data: dij input; t input; d_eij output; vij input; eta_eij output; d_eta_d_deij output
function [d_eij, eta_eij, d_eta_d_deij]   = fcn(dij, t, vij)

    d_eij = zeros(3,1);
    eta_eij = zeros(3,1);
    d_eta_d_deij = zeros(3,1);

    d12 = dij(1); d13 = dij(2); d14 = dij(3);
    v12 = vij(1); v13 = vij(2); v14 = vij(3);


    Omega_Hij = (2 - 0.1)*exp(-0.1*t) + 0.1;
    Omega_Wij = (1.8 - 0.1)*exp(-0.15*t) + 0.1;

    A = @(d_eij) (Omega_Hij*Omega_Wij*(Omega_Hij*Omega_Wij + d_eij^2))/((Omega_Hij - d_eij)^2*(Omega_Wij + d_eij)^2);

    d_e12 = d12 - v12; d_e13 = d13 - v13; d_e14 = d14 - v14;

    eta_e12 = (Omega_Hij*Omega_Wij*d_e12)/((Omega_Hij - d_e12) * (Omega_Wij + d_e12));
    eta_e13 = (Omega_Hij*Omega_Wij*d_e13)/((Omega_Hij - d_e13) * (Omega_Wij + d_e13));
    eta_e14 = (Omega_Hij*Omega_Wij*d_e14)/((Omega_Hij - d_e14) * (Omega_Wij + d_e14));

    d_eij = [d_e12; d_e13; d_e14];
    eta_eij = [eta_e12; eta_e13; eta_e14];

    d_eta_d_de12 = A(d_e12); d_eta_d_de13 = A(d_e13); d_eta_d_de14 = A(d_e14);

    d_eta_d_deij = [d_eta_d_de12; d_eta_d_de13; d_eta_d_de14];
    
end

== matlab function Pay_load/UAV3 Controller/Subsystem1/Position Controller/MATLAB Function1 ==
  data: dei input; eta_ei input; d_eta_d_dei input; ei input; eij input; d_ij input; Ei output; eta_eij input; d_eta_d_eij input
function Ei = fcn(dei, eta_ei, d_eta_d_dei, ei, eij, d_ij, eta_eij, d_eta_d_eij)

    Ei = zeros(3,1);

    A = d_eta_d_dei * sqrt(d_eta_d_dei) * ei;
    
    B = zeros(3,1);
    for i = 1:3
        B = B + 2*eta_eij(i)*d_eta_d_eij(i)*eij(((i-1)*3+1):(i*3),1)/d_ij(i);
    end

    Ei = A + B;

end

== matlab function Pay_load/Subsystem2/UAV3/MATLAB Function1 ==
  data: tau input; omega_dot output; omega input; Iv parameter
function omega_dot = fcn(tau, omega, Iv)
    
    omega_dot = zeros(3,1);

    omega_dot = Iv \ (tau - cross(omega, Iv*omega));

end

== matlab function Pay_load/UAV3 Controller/Subsystem1/Subsystem/MATLAB Function ==
  data: pi input; vi input; ui output; alpha_pi input; alpha_pi_dot input; Ei input; cable_tension input; delta_i input; rho_mi input; xL input; z2i output; ubar_i output; delta_i_dot output; rho_mi_dot output; m parameter; ri parameter
function [ui, z2i, ubar_i, delta_i_dot, rho_mi_dot] = ...
    Velocity_Control_41_44(pi, vi, alpha_pi, alpha_pi_dot, Ei, ...
                          cable_tension, delta_i, rho_mi, xL, m, ri)
    %#codegen
    % Vector inputs: 3x1
    % mi, delta_i, rho_mi: scalar
    
    K2i       = 3.15;
    epsilon_i = 0.1;
    
    n_delta     = 0.15;
    sigma_delta = 0.05;
    
    n_rho_m     = 0.1;
    sigma_rho_m = 0.01;
    
    assert(m > 0);
    
    ez = [0; 0; 1];
    
    z2i = vi - alpha_pi;
    z2_sq = z2i.' * z2i;
    
    %% Equation (42)
    pL = xL(1:3,1); phi_L = xL(7,1); theta_L = xL(8,1); psi_L = xL(9,1);

    RL = [cos(theta_L)*cos(psi_L), sin(phi_L)*sin(theta_L)*cos(psi_L) - cos(phi_L)*sin(psi_L), cos(phi_L)*sin(theta_L)*cos(psi_L) + sin(phi_L)*sin(psi_L);
          cos(theta_L)*sin(psi_L), sin(phi_L)*sin(theta_L)*sin(psi_L) + cos(phi_L)*cos(psi_L), cos(phi_L)*sin(theta_L)*sin(psi_L) - sin(phi_L)*cos(psi_L);
          -sin(theta_L), sin(phi_L)*cos(theta_L), cos(phi_L)*cos(theta_L)];

    qi = RL.'*(pL + RL*ri - pi)/norm(pL + RL*ri - pi);

    fCablePred_i = RL*qi*(cable_tension.'*qi);

    ubar_i = Ei - alpha_pi_dot ...
             + 9.81 * ez ...
             + K2i * z2i ...
             + delta_i * z2i / sqrt(z2_sq + epsilon_i^2) ...
             + fCablePred_i / m;
    
    %% Equation (41)
    ubar_sq = ubar_i.' * ubar_i;
    A = ubar_sq * rho_mi^2;
    
    ui = z2i * A / sqrt(z2_sq * A + epsilon_i^2);
    
    %% Equation (43)
    delta_i_dot = n_delta * z2_sq ...
                  / sqrt(z2_sq + epsilon_i^2) ...
                  - sigma_delta * delta_i;
    
    %% Equation (44)
    rho_mi_dot = n_rho_m * (z2i.' * ubar_i) ...
                - sigma_rho_m * rho_mi;

end

== matlab function Pay_load/UAV3 Controller/Subsystem1/Subsystem/MATLAB Function1 ==
  data: ui input; Fi output; psi_di input; angle_di_prev input; angle_di output; valid output
function [Fi, angle_di, valid] = ...
    Desired_Attitude_85_87(ui, psi_di, angle_di_prev)
%#codegen
% ui, angle_di_prev: 3x1
% psi_di, Fi: scalar
% valid: boolean

Fmin = 1e-8;

Fi = norm(ui);
angle_di = angle_di_prev;
valid = false;

% Khi ui gan 0, huong luc khong xac dinh.
% Giu goc dat truoc do, khong chia cho Fi.
if Fi <= Fmin
    return;
end

% Mien Euler bay thang dang su dung:
% |phi_di| < pi/2, |theta_di| < pi/2.
% assert(ui(3) > 0);

sphi = (ui(1)*sin(psi_di) ...
        - ui(2)*cos(psi_di)) / Fi;

% Chi chan sai so lam tron cua asin.
sphi = min(1.0, max(-1.0, sphi));

phi_di = asin(sphi);

theta_di = atan2( ...
    ui(1)*cos(psi_di) + ui(2)*sin(psi_di), ui(3));

angle_di = [phi_di; theta_di; psi_di];
valid = true;

end

== matlab function Pay_load/UAV4 Controller/Subsystem/MATLAB Function ==
  data: angle_i input; z3i output size=[3,1]; omega_i input; angle_di input; z4i output size=[3,1]; Gamma_i output size=[3,3]; alpha_angle_i output size=[3,1]; angle_i_dot output size=[3,1]; Psi_i output size=[3,3]; Psi_i_dot output size=[3,3]
function [z3i, z4i, Gamma_i, alpha_angle_i, angle_i_dot, Psi_i, Psi_i_dot] = ...
    Attitude_Error_56(angle_i, omega_i, angle_di)


    K3i = 0.75;
    nu_i = 0.5;
    
    phi   = angle_i(1);
    theta = angle_i(2);
    
    sp = sin(phi);
    cp = cos(phi);
    st = sin(theta);
    ct = cos(theta);
    
    assert(K3i > 0 && nu_i > 0);
    assert(abs(ct) > 1e-6);
    
    Gamma_i = [1, sp*st/ct, cp*st/ct;
               0, cp,       -sp;
               0, sp/ct,    cp/ct];
    
    Psi_i = [1, 0,   -st;
             0, cp,  sp*ct;
             0, -sp, cp*ct];
    
    angle_i_dot = Gamma_i * omega_i;
    
    z3i = angle_i - angle_di;
    
    k = K3i + 0.5*nu_i;
    alpha_angle_i = -k * z3i;
    
    z4i = angle_i_dot - alpha_angle_i;
    
    % Dao ham giai tich cua Psi_i
    phi_dot   = angle_i_dot(1);
    theta_dot = angle_i_dot(2);
    
    Psi_i_dot = ...
        [0, 0, -ct*theta_dot;
         0, -sp*phi_dot, ...
            cp*ct*phi_dot - sp*st*theta_dot;
         0, -cp*phi_dot, ...
            -sp*ct*phi_dot - cp*st*theta_dot];

end

== matlab function Pay_load/UAV4 Controller/Subsystem/MATLAB Function1 ==
  data: alpha_angle_i input; angle_i_dot input; Psi_i input; Xi_i output size=1; Psi_i_dot input
function Xi_i = Xi_89(alpha_angle_i, angle_i_dot, Psi_i, Psi_i_dot)

K3i = 0.75; nu_i = 0.5;

k = K3i + 0.5*nu_i;

w = Psi_i * angle_i_dot;

S_w = [0,    -w(3),  w(2);
       w(3),  0,    -w(1);
      -w(2),  w(1),  0];

term1 = norm(Psi_i_dot * alpha_angle_i);
term2 = norm(k * Psi_i * angle_i_dot);
term3 = norm(S_w, 2) * norm(Psi_i * alpha_angle_i);
term4 = norm(k * Psi_i, 2);

Xi_i = norm(Psi_i, 2) * (term1 + term2 + term3 + term4);

end

== matlab function Pay_load/UAV4 Controller/Subsystem/MATLAB Function2 ==
  data: z3i input; tau_i output; z4i input; Gamma_i input; Psi_i input; Xi_i input; rho_Ji input; zeta_i input; tau_bar_i output; rho_Ji_dot output; zeta_i_dot output
function [tau_i, tau_bar_i, rho_Ji_dot, zeta_i_dot] = ...
    Torque_Control_58_61(z3i, z4i, Gamma_i, Psi_i, ...
                         Xi_i, rho_Ji, zeta_i)
%#codegen
% z3i, z4i, tau_i, tau_bar_i: 3x1
% Gamma_i, Psi_i: 3x3
% Other inputs and adaptive derivatives: scalar

epsilon_i = 0.1;

n_rho_J     = 0.15;
sigma_rho_J = 0.05;

n_zeta     = 0.15;
sigma_zeta = 0.05;

K4i = 0.75;

assert(K4i > 0);

z4_sq = z4i.' * z4i;
Xi_sq = Xi_i^2;

den_zeta = sqrt(z4_sq * Xi_sq + epsilon_i^2);

% Equation (59)
GammaT_z4 = Gamma_i.' * z4i;

tau_bar_i = K4i * GammaT_z4 ...
            + Gamma_i.' * z3i ...
            + zeta_i * GammaT_z4 * Xi_sq / den_zeta;

% Equation (58)
q = Psi_i * z4i;

tau_bar_sq = tau_bar_i.' * tau_bar_i;
A = tau_bar_sq * rho_Ji^2;

tau_i = -q * A / sqrt((q.' * q) * A + epsilon_i^2);

% Equation (60)
rho_Ji_dot = n_rho_J * (q.' * tau_bar_i) ...
            - sigma_rho_J * rho_Ji;

% Equation (61)
zeta_i_dot = n_zeta * z4_sq * Xi_sq / den_zeta ...
            - sigma_zeta * zeta_i;

end

== matlab function Pay_load/UAV4 Controller/Subsystem1/Position Controller/Equation (10) ==
  data: e41 input; dij output; e42 input; e43 input
function dij = fcn(e41, e42, e43)

    dij = zeros(3,1);

    d41 = norm(e41);
    d42 = norm(e42);
    d43 = norm(e43);


    dij = [d41; d42; d43];
end

== matlab function Pay_load/UAV4 Controller/Subsystem1/Position Controller/Equation (15) ==
  data: dei input; eta_e4 output; t input; d_eta_d_dei output
function [eta_e4, d_eta_d_dei]= fcn(dei, t)
    
    eta_e4 = 0;

    Omega_dHi = (7.8 - 0.2)*exp(-0.4*t) + 0.2;

    eta_e4 = (Omega_dHi*dei)/(Omega_dHi - dei);

    d_eta_d_dei = Omega_dHi^2/(Omega_dHi - dei)^2;

end

== matlab function Pay_load/Subsystem3/UAV4/MATLAB Function ==
  data: a_free input; p_ddot output; fCableWorld input; m parameter
function p_ddot = UAV_Acceleration(a_free, fCableWorld, m)
%#codegen
% fCableWorld: luc day THUC tac dung len UAV, he the gioi.

assert(m > 0);

p_ddot = a_free + fCableWorld/m;
end

== matlab function Pay_load/UAV4 Controller/Subsystem1/Position Controller/Equation (38) ==
  data: ei input; dei input; eta_ei input; d_eta_d_dei input; alpha_pi output; Ei input; eta_eij input; pd_dot input; t input; e_dij input; e_dij_dot input; vij input; d_eij input; d_eta_d_deij input
function alpha_pi = fcn(ei, dei, eta_ei, d_eta_d_dei, Ei, eta_eij, pd_dot, t, e_dij, e_dij_dot, vij, d_eij, d_eta_d_deij)

    alpha_pi = zeros(3,1);

    Kei = 3.15; Keij = 0.45;
    
    %% Eta_i
    Omega_dHi = (7.8 - 0.2)*exp(-0.4*t) + 0.2;
    Omega_dHi_dot = -0.4*7.6*exp(-0.4*t);
    d_eta_d_Omega_dHi = -dei^2/(Omega_dHi - dei)^2;

    h = Omega_dHi;
    hdot = Omega_dHi_dot;
    gap = h - dei;

    assert(gap > 1e-9, ...
        'Sai so vi tri da cham hoac vuot bien.');

    Gi = (h/gap)^3 * ei;

    eta_Eta_i = Gi.'*pd_dot ...
                + eta_ei*(dei^2/gap^2)*hdot;
    
    
    %% Eta_eij
    Omega_Hij = (2 - 0.1)*exp(-0.1*t) + 0.1;
    Omega_Wij = (1.8 - 0.1)*exp(-0.15*t) + 0.1;

    Omega_Hij_dot = -0.1*1.9*exp(-0.1*t);
    Omega_Wij_dot = -0.15*1.7*exp(-0.15*t);

    C_Hij = @(d_eij) -Omega_Wij*d_eij^2/((Omega_Hij - d_eij)^2 * (Omega_Wij + d_eij));
    D_Wij = @(d_eij) Omega_Hij*d_eij^2/((Omega_Hij - d_eij)*(Omega_Wij + d_eij)^2);

    d_eta_d_Omega_Hij = [C_Hij(d_eij(1)); C_Hij(d_eij(2)); C_Hij(d_eij(3))];
    d_eta_d_Omega_Wij = [D_Wij(d_eij(1)); D_Wij(d_eij(2)); D_Wij(d_eij(3))];


    e_d12 = e_dij(1:3,1); e_d13 = e_dij(4:6,1); e_d14 = e_dij(7:9,1);
    e_d12_dot = e_dij_dot(1:3,1); e_d13_dot = e_dij_dot(4:6,1); e_d14_dot = e_dij_dot(7:9,1);
    
    Eta_e12 = d_eta_d_deij(1)/vij(1)*(e_d12(1)*e_d12_dot(1) + e_d12(2)*e_d12_dot(2) + e_d12(3)*e_d12_dot(3)) - (d_eta_d_Omega_Hij(1)*Omega_Hij_dot + d_eta_d_Omega_Wij(1)*Omega_Wij_dot);
    Eta_e13 = d_eta_d_deij(2)/vij(2)*(e_d13(1)*e_d13_dot(1) + e_d13(2)*e_d13_dot(2) + e_d13(3)*e_d13_dot(3)) - (d_eta_d_Omega_Hij(2)*Omega_Hij_dot + d_eta_d_Omega_Wij(2)*Omega_Wij_dot);
    Eta_e14 = d_eta_d_deij(3)/vij(3)*(e_d14(1)*e_d14_dot(1) + e_d14(2)*e_d14_dot(2) + e_d14(3)*e_d14_dot(3)) - (d_eta_d_Omega_Hij(3)*Omega_Hij_dot + d_eta_d_Omega_Wij(3)*Omega_Wij_dot);

    Eta_eij = [Eta_e12; Eta_e13; Eta_e14];

    B = 0;
    for i = 1:3
        B = B - Keij*eta_eij(i)^2 + eta_eij(i)*Eta_eij(i);
    end

    den = Ei.'*Ei;

    assert(den > 1e-12, ...
        'Phuong trinh 38 gan ky di: Ei gan bang 0.');

    alpha_pi = Ei/den * ...
            (-Kei*eta_ei^2 + eta_Eta_i + B);

end

== matlab function Pay_load/UAV4 Controller/Subsystem1/Position Controller/Equation (8) ==
  data: ei input; dei output
function dei = fcn(ei)

    dei = norm(ei);

end

== matlab function Pay_load/UAV4 Controller/Subsystem1/Position Controller/Equation (9) ==
  data: e_d41 input; vij output; e_d42 input; e_d43 input
function vij = fcn(e_d41, e_d42, e_d43)

    vij = zeros(3,1);

    v41 = norm(e_d41);
    v42 = norm(e_d42);
    v43 = norm(e_d43);

    vij = [v41; v42; v43];

end

== matlab function Pay_load/UAV4 Controller/Subsystem1/Position Controller/MATLAB Function ==
  data: dij input; t input; d_eij output; vij input; eta_eij output; d_eta_d_deij output
function [d_eij, eta_eij, d_eta_d_deij]   = fcn(dij, t, vij)

    d_eij = zeros(3,1);
    eta_eij = zeros(3,1);
    d_eta_d_deij = zeros(3,1);

    d12 = dij(1); d13 = dij(2); d14 = dij(3);
    v12 = vij(1); v13 = vij(2); v14 = vij(3);


    Omega_Hij = (2 - 0.1)*exp(-0.1*t) + 0.1;
    Omega_Wij = (1.8 - 0.1)*exp(-0.15*t) + 0.1;

    A = @(d_eij) (Omega_Hij*Omega_Wij*(Omega_Hij*Omega_Wij + d_eij^2))/((Omega_Hij - d_eij)^2*(Omega_Wij + d_eij)^2);

    d_e12 = d12 - v12; d_e13 = d13 - v13; d_e14 = d14 - v14;

    eta_e12 = (Omega_Hij*Omega_Wij*d_e12)/((Omega_Hij - d_e12) * (Omega_Wij + d_e12));
    eta_e13 = (Omega_Hij*Omega_Wij*d_e13)/((Omega_Hij - d_e13) * (Omega_Wij + d_e13));
    eta_e14 = (Omega_Hij*Omega_Wij*d_e14)/((Omega_Hij - d_e14) * (Omega_Wij + d_e14));

    d_eij = [d_e12; d_e13; d_e14];
    eta_eij = [eta_e12; eta_e13; eta_e14];

    d_eta_d_de12 = A(d_e12); d_eta_d_de13 = A(d_e13); d_eta_d_de14 = A(d_e14);

    d_eta_d_deij = [d_eta_d_de12; d_eta_d_de13; d_eta_d_de14];
    
end
